simulink subsystem "Engine_refsub_Basic"  (R2023a)
settings: Solver=VariableStepAuto  StartTime=0.0  StopTime=10.0  RelTol=1e-3
undefined symbols (not defined in the file or in its folder): engine
libraries: fl_lib x9, nesl_utility x4, sdl_lib x2
settings Model: Creator=isaacito  LastModifiedBy=isaacito
settings SolverCC: AlgebraicLoopSolver=TrustRegion
settings OptimizationCC: ReuseModelBlockBuffer=off
settings DebuggingCC: UnconnectedInputMsg=warning  UnconnectedOutputMsg=warning  UnconnectedLineMsg=warning
settings ModelReferenceCC: EnableRefExpFcnMdlSchedulingChecks=on
settings RTWCC: DLArmComputeVersion=19.05

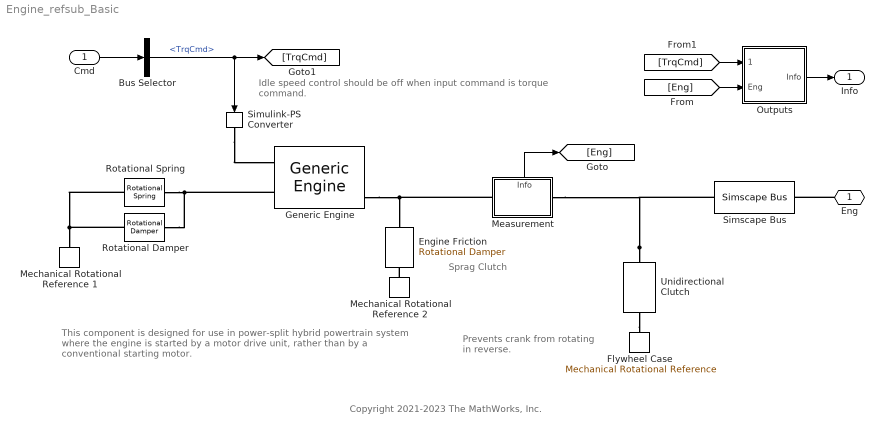
== system Engine_refsub_Basic ==
  note: This component is designed for use in
      | power-split hybrid powertrain system where
      | the engine is started by a motor drive unit,
      | rather than by a conventional starting motor.
  note: Copyright 2021-2023 The MathWorks, Inc.
  note: Sprag Clutch
  note: Prevents crank from
      | rotating in reverse.
  note: Idle speed control should be off
      | when input command is torque command.
  Cmd : Inport
  Bus Selector : BusSelector  OutputSignals=TrqCmd
  Engine Friction : fl_lib/Mechanical/Rotational Elements/Rotational Damper  D=engine.damping_Nm_per_rpm m*N/rpm  w_specify=off  w_priority=None  w=0 rad/s  w_nominal_specify=off  w_nominal_unit=rad/s  w_nominal_value=1  t_specify=off  t_priority=None  t=0 N*m  t_nominal_specify=off  t_nominal_unit=N*m  t_nominal_value=1
  Flywheel Case : fl_lib/Mechanical/Rotational Elements/Mechanical Rotational Reference
  Generic Engine : sdl_lib/Engines & Motors/Generic Engine  input_type=sdl.enum.GenericEngineInputType.TorqueCommand  model_parameterization=sdl.enum.engineParameterization.polynomial  engine_type=sdl.enum.engineType.Generic  Trq_max=engine.trqMax_Nm N*m  w_Trq_max=engine.trqMaxSpd_rpm rpm  P_max=engine.powerMax_kW kW  w_P_max=6858 rpm  w_max=engine.maxSpd_rpm rpm  w_min=engine.stallSpd_rpm rpm  w_tab=[500, 1000, 2000, 3000, 4300, 5000, 6000, 7000] rpm  trq_tab=[250, 280, 330, 360, 380, 370, 350, 310] N*m  pwr_tab=[10, 30, 70, 110, 165, 190, 220, 230] kW  interp_method=simscape.enum.interpolation.linear  w_thr=engine.smoothing_rpm rpm  model_inertia=sdl.enum.model_inertia.on  inertia=engine.inertia_kg_m2 kg*m^2  initial_velocity=initial.engine_speed_rpm rpm  model_time_constant=sdl.enum.lagOffOn.off  time_constant=engine.lag_s s  initial_normalized_throttle=0  fc_model=sdl.enum.fuel_consumption_model.FuelOff  fc_per_rev=25 mg/rev  fc_w_tab=[1000, 2000, 3000, 4000, 5000, 6000] rpm  fc_trq_tab=[0, 80, 160, 200, 240, 320, 360, 400] N*m  fc_tab=[.5, .9, 1.4, 1.6, 1.9, 2.7, 3.4, 4.4; 1, 1.7, 2.7, 3.1, 3.6, 5, 6, 7.4; 1.4, 2.7, 4, 4.8, 5.6, 7.5, 8.5, 10.5; 2, 3.6, 5.8, 6.7, 8, 10.4, 11.7, 13.3; 2.5, 4.8, 7.9, 9.4, 10.8, 14, 16.2, 18.6; 3.1, 6, 10.3, 11.9, 13.8, 18.4, 22, 26.5] g/s  bmep_tab=[0, 250, 500, 625, 750, 1000, 1150, 1250] kPa  bsfc_tab=[410, 380, 300, 280, 270, 290, 320, 380; 410, 370, 290, 270, 260, 270, 285, 320; 415, 380, 290, 275, 265, 270, 270, 300; 420, 390, 310, 290, 285, 280, 280, 285; 430, 410, 340, 320, 310, 300, 310, 320; 450, 430, 370, 340, 330, 330, 350, 380] g/(hr*kW)  fc_interp_method=simscape.enum.interpolation.linear  displaced_volume=400 cm^3  rev_per_cycle=2  idle_speed=false  idle_speed_reference=1000 rpm  tau_controller=1 s  idle_w_thr=1 rpm  redline=false  redline_speed=5000 rpm  tau_redline=1 s  redline_w_thr=1 rpm
      settings: InternalSimscapePortConfiguration="{\"Bottom\":[],\"Left\":[{\"id\":\"TrqCmd\",\"label\":\"Trq\",\"type\":\"input\"},{\"id\":\"B\",\"label\":\"B\",\"type\":\"foundation.mechanical.rotational.rotational\"}],\"Right\":[{\"id\":\"P\",\"label\":\"P\",\"type\":\"output\"},{\"id\":\"FC\",\"label\":\"FC\",\"type\":\"output\"},{\"id\":\"F\",\"label\":\"F\",\"type\":\"foundation.mechanical.rotational.rotational\"}],\"Top\":[]}"
  Measurement : Subsystem
      settings: PortSchema="{\"entries\":[{\"content\":{\"sides\":[{\"content\":{\"connectorIds\":[\"LConn1\"]},\"type\":\"ConnectorPlacement.EquallySpacedRectSide\",\"uuid\":\"07c2ae95-e870-4b8d-a90d-f6f29bd91438\"},{\"content\":{\"connectorIds\":[\"RConn1\"],\"side\":\"RIGHT\"},\"type\":\"ConnectorPlacement.EquallySpacedRectSide\",\"uuid\":\"a6bad6b4-02de-43bd-83c0-90c7caa8debd\"},{\"content\":{\"connectorIds\":[\"Out1\"],\"side\":\"TOP\"},\"type\":\"ConnectorPlacement.EquallySpacedRectSide\",\"uuid\":\"e2b5c796-e9a6-4d01-87a6-78788a72fccc\"}]},\"type\":\"ConnectorPlacement.EquallySpacedConnector\",\"uuid\":\"494e0008-7a6b-45d1-a26f-72f06cc564cf\"}],\"packageUris\":[\"http://schema.mathworks.com/mf0/Connector/R2020b\"],\"version\":\"1.0\"}"
  Mechanical Rotational Reference 1 : fl_lib/Mechanical/Rotational Elements/Mechanical Rotational Reference
  Mechanical Rotational Reference 2 : fl_lib/Mechanical/Rotational Elements/Mechanical Rotational Reference
  Outputs : Subsystem
  Rotational Damper : fl_lib/Mechanical/Rotational Elements/Rotational Damper  D=engine.dampSpringFriction_Nm_per_rpm N*m/rpm  w_specify=off  w_priority=None  w=0 rad/s  w_nominal_specify=off  w_nominal_unit=rad/s  w_nominal_value=1  t_specify=off  t_priority=None  t=0 N*m  t_nominal_specify=off  t_nominal_unit=N*m  t_nominal_value=1
  Rotational Spring : fl_lib/Mechanical/Rotational Elements/Rotational Spring  spr_rate=engine.dampSpringStiffness_Nm_per_rad N*m/rad  w_specify=off  w_priority=None  w=0 rad/s  w_nominal_specify=off  w_nominal_unit=rad/s  w_nominal_value=1  t_specify=off  t_priority=None  t=0 N*m  t_nominal_specify=off  t_nominal_unit=N*m  t_nominal_value=1  phi_specify=on  phi_priority=Low  phi=0 rad  phi_nominal_specify=off  phi_nominal_unit=rad  phi_nominal_value=1
      settings: AttributesFormatString=Deformation priority: %<phi_priority>
  Simscape Bus : SimscapeBus  HierarchyStrings=AngSpd  ConnectionType=Bus: Bus_Rotational
      settings: AttributesFormatString=%<ConnectionType>
  Simulink-PS Converter : nesl_utility/Simulink-PS Converter  PhysicalDomain=network_engine_domain  SubClassName=ps_input  LeftPortType=input  RightPortType=output  PseudoPeriodic=off  Frequencies=[]  NoiseDistribution=none  NoiseParameters=[]  Unit=N*m  AffineConversion=off  FilteringAndDerivatives=provide  SimscapeFilterOrder=1  InputFilterTimeConstant=0.001  UdotUserProvided=0
  Unidirectional Clutch : sdl_lib/Clutches/Unidirectional Clutch  transmission_direction=2  initial_state_locked=sdl.enum.initial_lock.unlocked
      settings: AttributesFormatString=%<initial_state_locked>  InternalSimscapePortConfiguration="{\"Bottom\":[],\"Left\":[{\"id\":\"H\",\"label\":\"H\",\"type\":\"foundation.mechanical.rotational.rotational\"}],\"Right\":[{\"id\":\"R\",\"label\":\"R\",\"type\":\"foundation.mechanical.rotational.rotational\"}],\"Top\":[]}"
  Eng : PMIOPort  Side=Left
  Info : Outport
  wires:
  Measurement/1(Info) -> [Eng]
  [TrqCmd] -> Outputs/1(TrqCmd)
  [Eng] -> Outputs/2(Eng)
  Bus Selector/1 -> [TrqCmd], Simulink-PS Converter/1  "<TrqCmd>"
  Cmd/1 -> Bus Selector/1
  Outputs/1(Info) -> Info/1
  connections:
  Rotational Spring/RConn1 -- Rotational Damper/RConn1 -- Generic Engine/LConn2
  Rotational Spring/LConn1 -- Rotational Damper/LConn1 -- Mechanical Rotational Reference 1/LConn1
  Measurement/LConn1 -- Generic Engine/RConn3 -- Engine Friction/LConn1
  Unidirectional Clutch/LConn1 -- Measurement/RConn1 -- Simscape Bus/LConn1
  Unidirectional Clutch/RConn1 -- Flywheel Case/LConn1
  Mechanical Rotational Reference 2/LConn1 -- Engine Friction/RConn1
  Simulink-PS Converter/RConn1 -- Generic Engine/LConn1
  Eng/RConn1 -- Simscape Bus/RConn1

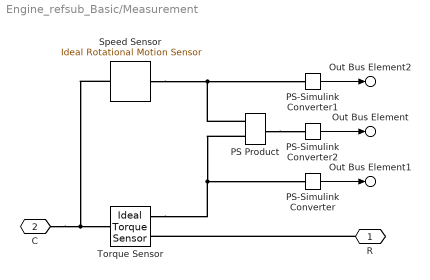
== system Engine_refsub_Basic/Measurement ==
  PS Product : fl_lib/Physical Signals/Functions/PS Product
  PS-Simulink Converter : nesl_utility/PS-Simulink Converter  PhysicalDomain=network_engine_domain  SubClassName=ps_output  LeftPortType=input  RightPortType=output  PseudoPeriodic=off  Frequencies=[]  VectorFormat=1-D array  Unit=N*m  AffineConversion=off
  PS-Simulink Converter1 : nesl_utility/PS-Simulink Converter  PhysicalDomain=network_engine_domain  SubClassName=ps_output  LeftPortType=input  RightPortType=output  PseudoPeriodic=off  Frequencies=[]  VectorFormat=1-D array  Unit=rpm  AffineConversion=off
  PS-Simulink Converter2 : nesl_utility/PS-Simulink Converter  PhysicalDomain=network_engine_domain  SubClassName=ps_output  LeftPortType=input  RightPortType=output  PseudoPeriodic=off  Frequencies=[]  VectorFormat=1-D array  Unit=kW  AffineConversion=off
  Speed Sensor : fl_lib/Mechanical/Mechanical Sensors/Ideal Rotational Motion Sensor  reference=foundation.enum.MeasurementReference.absolute  acceleration_port=false  velocity_port=true  position_port=false  wrap_angle=simscape.enum.onoff.off  offset=0 rad
      settings: InternalSimscapePortConfiguration="{\"Bottom\":[],\"Left\":[{\"id\":\"R\",\"label\":\"R\",\"type\":\"foundation.mechanical.rotational.rotational\"}],\"Right\":[{\"id\":\"W\",\"label\":\"W\",\"type\":\"output\"}],\"Top\":[]}"
  Torque Sensor : fl_lib/Mechanical/Mechanical Sensors/Ideal Torque Sensor
  R : PMIOPort  Side=Right
  C : PMIOPort  Port=2  Side=Left
  Out Bus Element : Outport  PortName=Info  Element=EngPwr
  Out Bus Element1 : Outport  PortName=Info  Element=EngTrq
  Out Bus Element2 : Outport  PortName=Info  Element=EngSpd
  wires:
  PS-Simulink Converter1/1 -> Out Bus Element2/1
  PS-Simulink Converter/1 -> Out Bus Element1/1
  PS-Simulink Converter2/1 -> Out Bus Element/1
  connections:
  R/RConn1 -- Torque Sensor/RConn1
  Speed Sensor/LConn1 -- C/RConn1 -- Torque Sensor/LConn1
  PS Product/RConn1 -- PS-Simulink Converter2/LConn1
  PS Product/LConn2 -- Torque Sensor/RConn2 -- PS-Simulink Converter/LConn1
  Speed Sensor/RConn1 -- PS Product/LConn1 -- PS-Simulink Converter1/LConn1

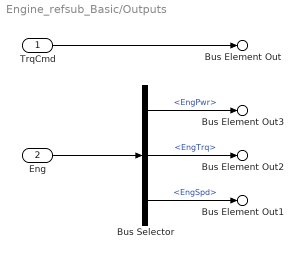
== system Engine_refsub_Basic/Outputs ==
  TrqCmd : Inport
  Eng : Inport  Port=2
  Bus Selector : BusSelector  OutputSignals=EngPwr,EngTrq,EngSpd
  Bus Element Out : Outport  PortName=Info  Element=EngTrqCmd
      settings: AttributesFormatString=%<Unit>
  Bus Element Out1 : Outport  PortName=Info  Element=EngSpd
      settings: AttributesFormatString=%<Unit>
  Bus Element Out3 : Outport  PortName=Info  Element=EngPwr
      settings: AttributesFormatString=%<Unit>
  Bus Element Out2 : Outport  PortName=Info  Element=EngTrq
      settings: AttributesFormatString=%<Unit>
  wires:
  Eng/1 -> Bus Selector/1
  Bus Selector/1 -> Bus Element Out3/1  "<EngPwr>"
  Bus Selector/2 -> Bus Element Out2/1  "<EngTrq>"
  TrqCmd/1 -> Bus Element Out/1
  Bus Selector/3 -> Bus Element Out1/1  "<EngSpd>"
